simulink model "inv_im_param"  (R2026b)
settings: Solver=ode23tb  StopTime=param.sim.simlength  FixedStep=tc  MaxStep=param.glb_time.tc
values from neighbouring files (symbols this model uses):
  param = add_template_extras(param, options)    [init_model.m]
undefined symbols (not defined in the file or in its folder): magnitude
libraries: fl_lib x30, nesl_utility x13, lithium_ion_battery x1, induction_machine x1, dclink_with_center_tap x1, dead_time_generator_cmos_simulink x1, three_phase_pwm_modulator x1, three_phase_inverter_ideal_switch_based_model x1, three_phase_inverter_igbt_advanced_thermal_model x1, three_phase_inverter_mosfet_based_with_thermal_model x1, threephase_inductor_lib x1, simple_flexible_shaft x1
(part 3 of 3)

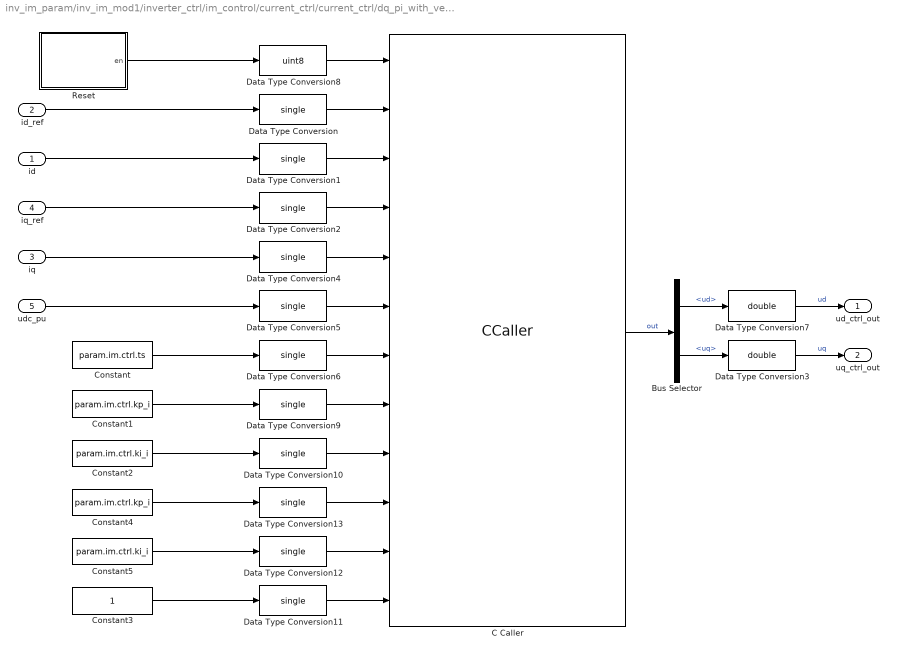
== system inv_im_param/inv_im_mod1/inverter_ctrl/im_control/current_ctrl/current_ctrl/dq_pi_with_vector_antiwindup mod1/dq_vector_pi_ccaller ==
  id : Inport
  id_ref : Inport  Port=2
  iq : Inport  Port=3
  iq_ref : Inport  Port=4
  udc_pu : Inport  Port=5
  Bus Selector : BusSelector  OutputSignals=ud,uq
  C Caller : CCaller  FunctionName=dqvector_pi_process_simulink  PortSpecificationStruct="%)30     .    ,!8   8    (     @         %    \"     T    !     0         %  0 \"0    $    _    07)G3F%M90  4&]R=$YA;64 4V-O<&4     26YD97@     5'EP90      4VEZ90      27-';&]B86P   X    P    !@    @    $          4    (     0    ,    !         !   P!O=70 #@   #     &    \"     0         !0    @    !     P    $         $  # &]U=  .    .     8    (    !          %    \"     $    &     0         0   ...(+7280 chars)"
  Constant : Constant  Value=param.im.ctrl.ts
  Constant1 : Constant  Value=param.im.ctrl.kp_i
  Constant2 : Constant  Value=param.im.ctrl.ki_i
  Constant3 : Constant
  Constant4 : Constant  Value=param.im.ctrl.kp_i
  Constant5 : Constant  Value=param.im.ctrl.ki_i
  Data Type Conversion{,1..2,4..6,9..13} (11 alike) : DataTypeConversion  OutDataTypeStr=single  SaturateOnIntegerOverflow=off  RndMeth=Floor
  Data Type Conversion3 : DataTypeConversion  OutDataTypeStr=double  SaturateOnIntegerOverflow=off  RndMeth=Floor
  Data Type Conversion7 : DataTypeConversion  OutDataTypeStr=double  SaturateOnIntegerOverflow=off  RndMeth=Floor
  Data Type Conversion8 : DataTypeConversion  OutDataTypeStr=uint8  SaturateOnIntegerOverflow=off  RndMeth=Floor
  Reset : Subsystem
  ud_ctrl_out : Outport
  uq_ctrl_out : Outport  Port=2
  wires:
  Data Type Conversion5/1 -> C Caller/6
  Data Type Conversion/1 -> C Caller/2
  C Caller/1 -> Bus Selector/1  "out"
  Data Type Conversion1/1 -> C Caller/3
  Data Type Conversion4/1 -> C Caller/5
  Data Type Conversion2/1 -> C Caller/4
  Data Type Conversion6/1 -> C Caller/7
  Bus Selector/2 -> Data Type Conversion3/1  "<uq>"
  Bus Selector/1 -> Data Type Conversion7/1  "<ud>"
  Data Type Conversion7/1 -> ud_ctrl_out/1  "ud"
  Data Type Conversion3/1 -> uq_ctrl_out/1  "uq"
  Data Type Conversion8/1 -> C Caller/1
  Data Type Conversion9/1 -> C Caller/8
  Data Type Conversion10/1 -> C Caller/9
  Data Type Conversion11/1 -> C Caller/12
  Data Type Conversion13/1 -> C Caller/10
  Data Type Conversion12/1 -> C Caller/11
  Constant3/1 -> Data Type Conversion11/1
  Constant5/1 -> Data Type Conversion12/1
  Constant4/1 -> Data Type Conversion13/1
  Constant2/1 -> Data Type Conversion10/1
  Constant1/1 -> Data Type Conversion9/1
  Constant/1 -> Data Type Conversion6/1
  udc_pu/1 -> Data Type Conversion5/1
  iq/1 -> Data Type Conversion4/1
  iq_ref/1 -> Data Type Conversion2/1
  Reset/1(en) -> Data Type Conversion8/1
  id_ref/1 -> Data Type Conversion/1
  id/1 -> Data Type Conversion1/1

== system inv_im_param/inv_im_mod1/inverter_ctrl/im_control/current_ctrl/rotor_flux_estimators/ekf/extended_kalman_observer ==
  ualphabeta : Inport
  ialphabeta : Inport  Port=2
  udc_pu : Inport  Port=3
  ekf_im : MATLAB Function  TreatAsAtomicUnit=on
  ekf_state : Scope
      settings: ActiveDisplayYMinimum=-4.1303782529271533  ActiveDisplayYMaximum=2.0916402302067323  DataLoggingVariableName=ScopeData14
  voltage_delay : Delay  DelayLength=n_delay_u
  psi_alpha_ekf_hat : Outport
  psi_beta_ekf_hat : Outport  Port=2
  phase_elec_ekf_hat : Outport  Port=3
  omega_elec_ekf_hat : Outport  Port=4
  wires:
  ualphabeta/1 -> voltage_delay/1  "u_ab_cmd"
  voltage_delay/1 -> ekf_im/1(u_ab)  "u_ab"
  ialphabeta/1 -> ekf_im/2(i_ab)  "i_ab"
  udc_pu/1 -> ekf_im/3(udc_pu)  "udc_pu"
  ekf_im/1(psi_alpha) -> psi_alpha_ekf_hat/1  "psi_alpha"
  ekf_im/2(psi_beta) -> psi_beta_ekf_hat/1  "psi_beta"
  ekf_im/3(theta) -> phase_elec_ekf_hat/1  "theta"
  ekf_im/4(omega) -> omega_elec_ekf_hat/1  "omega"
  ekf_im/5(x_hat) -> ekf_state/1  "x(k|k)"

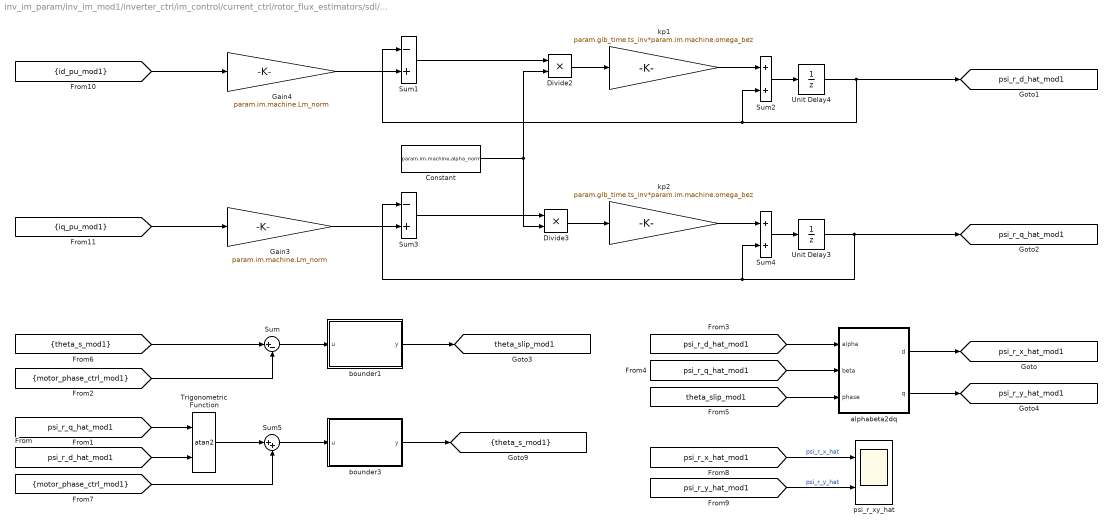
== system inv_im_param/inv_im_mod1/inverter_ctrl/im_control/current_ctrl/rotor_flux_estimators/sdl/observer_from_rotor ==
  Constant : Constant  Value=param.im.machine.alpha_norm
  Divide2 : Product
  Divide3 : Product
  Gain3 : Gain  Gain=param.im.machine.Lm_norm
  Gain4 : Gain  Gain=param.im.machine.Lm_norm
  Sum : Sum  Inputs=|+-
  Sum1 : Sum  Inputs=-+  SaturateOnIntegerOverflow=on
  Sum2 : Sum  SaturateOnIntegerOverflow=on
  Sum3 : Sum  Inputs=-+  SaturateOnIntegerOverflow=on
  Sum4 : Sum  SaturateOnIntegerOverflow=on
  Sum5 : Sum  Inputs=|++
  Trigonometric Function : Trigonometry  Operator=atan2
  Unit Delay3 : UnitDelay  SampleTime=-1
  Unit Delay4 : UnitDelay  SampleTime=-1
  alphabeta2dq : Subsystem
  bounder1 : MATLAB Function  TreatAsAtomicUnit=on
  bounder3 : MATLAB Function  TreatAsAtomicUnit=on
  kp1 : Gain  Gain=param.glb_time.ts_inv*param.im.machine.omega_bez  SaturateOnIntegerOverflow=on  OutDataTypeStr=Inherit: Same as input  ParamDataTypeStr=Inherit: Same as input
  kp2 : Gain  Gain=param.glb_time.ts_inv*param.im.machine.omega_bez  SaturateOnIntegerOverflow=on  OutDataTypeStr=Inherit: Same as input  ParamDataTypeStr=Inherit: Same as input
  psi_r_xy_hat : Scope  NumInputPorts=2
      settings: ActiveDisplayYMinimum=-0.0998429610041313  ActiveDisplayYMaximum=0.89858664903716645  DataLoggingVariableName=ScopeData10
  tag scope: psi_r_d_hat_mod1=global, psi_r_q_hat_mod1=global, psi_r_x_hat_mod1=global, psi_r_y_hat_mod1=global, theta_s_mod1=scoped, theta_slip_mod1=global
  wires:
  [psi_r_x_hat_mod1] -> psi_r_xy_hat/1  "psi_r_x_hat"
  bounder3/1(y) -> [theta_s_mod1]
  [psi_r_d_hat_mod1] -> Trigonometric Function/2
  Divide2/1 -> kp1/1
  bounder1/1(y) -> [theta_slip_mod1]
  Sum5/1 -> bounder3/1(u)
  Gain3/1 -> Sum3/2
  [psi_r_y_hat_mod1] -> psi_r_xy_hat/2  "psi_r_y_hat"
  [theta_s_mod1] -> Sum/1
  kp1/1 -> Sum2/1
  alphabeta2dq/2(q) -> [psi_r_y_hat_mod1]
  [iq_pu_mod1] -> Gain3/1
  Gain4/1 -> Sum1/2
  Unit Delay3/1 -> [psi_r_q_hat_mod1], Sum4/2, Sum3/1
  Unit Delay4/1 -> [psi_r_d_hat_mod1], Sum2/2, Sum1/1
  Divide3/1 -> kp2/1
  [theta_slip_mod1] -> alphabeta2dq/3(phase)
  Constant/1 -> Divide3/2, Divide2/2
  Sum4/1 -> Unit Delay3/1
  [motor_phase_ctrl_mod1] -> Sum/2
  Sum3/1 -> Divide3/1
  Trigonometric Function/1 -> Sum5/1
  kp2/1 -> Sum4/1
  alphabeta2dq/1(d) -> [psi_r_x_hat_mod1]
  Sum/1 -> bounder1/1(u)
  [psi_r_d_hat_mod1] -> alphabeta2dq/1(alpha)
  [id_pu_mod1] -> Gain4/1
  Sum2/1 -> Unit Delay4/1
  Sum1/1 -> Divide2/1
  [psi_r_q_hat_mod1] -> Trigonometric Function/1
  [motor_phase_ctrl_mod1] -> Sum5/2
  [psi_r_q_hat_mod1] -> alphabeta2dq/2(beta)

== system inv_im_param/inv_im_mod1/inverter_ctrl/im_control/current_ctrl/current_ctrl/dq_pi_with_vector_antiwindup mod1/dq_vector_pi/bounder1 ==
  md : Inport
  m_1 : Inport  Port=2
  m : Inport  Port=3
  Constant : Constant
  Constant1 : Constant  Value=0
  Divide : Product
  Switch : Switch  Threshold=1  SaturateOnIntegerOverflow=off  InputSameDT=off
  Switch1 : Switch  Threshold=1  SaturateOnIntegerOverflow=off  InputSameDT=off
  md_sat : Outport  VectorParamsAs1DForOutWhenUnconnected=off
  clip : Outport  Port=2  VectorParamsAs1DForOutWhenUnconnected=off
  wires:
  md/1 -> Switch1/3, Divide/2
  m_1/1 -> Divide/1
  Divide/1 -> Switch1/1
  Switch1/1 -> md_sat/1
  Switch/1 -> clip/1
  m/1 -> Switch/2, Switch1/2
  Constant/1 -> Switch/1
  Constant1/1 -> Switch/3

== system inv_im_param/inv_im_mod1/inverter_ctrl/im_control/current_ctrl/current_ctrl/dq_pi_with_vector_antiwindup mod1/dq_vector_pi/bounder2 ==
  m : Inport
  m_1 : Inport  Port=2
  mq : Inport  Port=3
  Constant : Constant
  Constant1 : Constant  Value=0
  Divide : Product
  Switch : Switch  Threshold=1  SaturateOnIntegerOverflow=off  InputSameDT=off
  Switch1 : Switch  Threshold=1  SaturateOnIntegerOverflow=off  InputSameDT=off
  mq_sat : Outport  VectorParamsAs1DForOutWhenUnconnected=off
  clip : Outport  Port=2  VectorParamsAs1DForOutWhenUnconnected=off
  wires:
  Constant1/1 -> Switch/3
  Constant/1 -> Switch/1
  m/1 -> Switch1/2, Switch/2
  Switch/1 -> clip/1
  Switch1/1 -> mq_sat/1
  Divide/1 -> Switch1/1
  m_1/1 -> Divide/1
  mq/1 -> Divide/2, Switch1/3

== system inv_im_param/inv_im_mod1/inverter_ctrl/im_control/current_ctrl/current_ctrl/dq_pi_with_vector_antiwindup mod1/dq_vector_pi/pi_d ==
  id_tilde : Inport
  clip : Inport  Port=2
  1/Ti : Gain  Gain=param.im.ctrl.kp_i  SaturateOnIntegerOverflow=on  OutDataTypeStr=Inherit: Same as input  ParamDataTypeStr=Inherit: Same as input
  Constant : Constant  Value=0
  Sum2 : Sum  Inputs=+-  SaturateOnIntegerOverflow=on
  Sum4 : Sum  SaturateOnIntegerOverflow=on
  Sum5 : Sum  SaturateOnIntegerOverflow=on
  Switch1 : Switch  Threshold=0.5  SaturateOnIntegerOverflow=off  InputSameDT=off
  Switch2 : Switch  Threshold=0.5  SaturateOnIntegerOverflow=off  InputSameDT=off
  Unit Delay1 : UnitDelay  SampleTime=-1
  Unit Delay2 : UnitDelay  SampleTime=-1
  kp1 : Gain  Gain=param.ctrl.CTRPIFF_CLIP_RELEASE*param.glb_time.ts_inv  SaturateOnIntegerOverflow=on  OutDataTypeStr=Inherit: Same as input  ParamDataTypeStr=Inherit: Same as input
  kp2 : Gain  Gain=param.im.ctrl.ki_i*param.glb_time.ts_inv  SaturateOnIntegerOverflow=on  OutDataTypeStr=Inherit: Same as input  ParamDataTypeStr=Inherit: Same as input
  ud_out : Outport  VectorParamsAs1DForOutWhenUnconnected=off
  wires:
  id_tilde/1 -> kp2/1, 1/Ti/1
  Sum5/1 -> ud_out/1
  Switch1/1 -> Unit Delay2/1
  Sum4/1 -> Sum5/2, Switch1/3
  kp1/1 -> Sum2/2
  Sum2/1 -> Switch1/1
  Unit Delay2/1 -> Sum4/2, kp1/1, Sum2/1
  1/Ti/1 -> Sum5/1
  Switch2/1 -> Sum4/1
  kp2/1 -> Switch2/3
  clip/1 -> Unit Delay1/1
  [clip] -> Switch2/2
  [clip] -> Switch1/2
  Constant/1 -> Switch2/1
  Unit Delay1/1 -> [clip]

== system inv_im_param/inv_im_mod1/inverter_ctrl/im_control/current_ctrl/current_ctrl/dq_pi_with_vector_antiwindup mod1/dq_vector_pi/pi_q ==
  iq_tilde : Inport
  clip : Inport  Port=2
  1/Ti : Gain  Gain=param.im.ctrl.kp_i  SaturateOnIntegerOverflow=on  OutDataTypeStr=Inherit: Same as input  ParamDataTypeStr=Inherit: Same as input
  Constant : Constant  Value=0
  Sum2 : Sum  Inputs=+-  SaturateOnIntegerOverflow=on
  Sum4 : Sum  SaturateOnIntegerOverflow=on
  Sum5 : Sum  SaturateOnIntegerOverflow=on
  Switch1 : Switch  Threshold=0.5  SaturateOnIntegerOverflow=off  InputSameDT=off
  Switch2 : Switch  Threshold=0.5  SaturateOnIntegerOverflow=off  InputSameDT=off
  Unit Delay1 : UnitDelay  SampleTime=-1
  Unit Delay2 : UnitDelay  SampleTime=-1
  kp1 : Gain  Gain=param.ctrl.CTRPIFF_CLIP_RELEASE*param.glb_time.ts_inv  SaturateOnIntegerOverflow=on  OutDataTypeStr=Inherit: Same as input  ParamDataTypeStr=Inherit: Same as input
  kp2 : Gain  Gain=param.im.ctrl.ki_i*param.glb_time.ts_inv  SaturateOnIntegerOverflow=on  OutDataTypeStr=Inherit: Same as input  ParamDataTypeStr=Inherit: Same as input
  Vqs_out : Outport  VectorParamsAs1DForOutWhenUnconnected=off
  wires:
  Constant/1 -> Switch2/1
  [clip] -> Switch1/2
  [clip] -> Switch2/2
  clip/1 -> Unit Delay1/1
  kp2/1 -> Switch2/3
  Switch2/1 -> Sum4/1
  1/Ti/1 -> Sum5/1
  Unit Delay2/1 -> Sum2/1, kp1/1, Sum4/2
  Sum2/1 -> Switch1/1
  kp1/1 -> Sum2/2
  Sum4/1 -> Sum5/2, Switch1/3
  Switch1/1 -> Unit Delay2/1
  iq_tilde/1 -> 1/Ti/1, kp2/1
  Unit Delay1/1 -> [clip]
  Sum5/1 -> Vqs_out/1

== system inv_im_param/inv_im_mod1/inverter_ctrl/im_control/current_ctrl/current_ctrl/dq_pi_with_vector_antiwindup mod1/dq_vector_pi/switch ==
  clip 1 : Inport
  clip 2 : Inport  Port=2
  Constant4 : Constant
  Constant5 : Constant  Value=0
  Sum1 : Sum  SaturateOnIntegerOverflow=on
  Switch : Switch  Threshold=0.5  SaturateOnIntegerOverflow=off  InputSameDT=off
  clip : Outport  VectorParamsAs1DForOutWhenUnconnected=off
  wires:
  Constant5/1 -> Switch/3
  Switch/1 -> clip/1
  Constant4/1 -> Switch/1
  Sum1/1 -> Switch/2
  clip 1/1 -> Sum1/1
  clip 2/1 -> Sum1/2

== system inv_im_param/inv_im_mod1/inverter_ctrl/im_control/current_ctrl/current_ctrl/dq_pi_with_vector_antiwindup mod1/dq_vector_pi/vector lenght ==
  md : Inport
  mq : Inport  Port=2
  Math Function : Math  Operator=magnitude^2  SignedPower=on
  Math Function1 : Math  Operator=magnitude^2  SignedPower=on
  Math Function2 : Math  Operator=reciprocal  SignedPower=on
  Sqrt : Sqrt
  Sum5 : Sum  SaturateOnIntegerOverflow=on
  m_1 : Outport  VectorParamsAs1DForOutWhenUnconnected=off
  m : Outport  Port=2  VectorParamsAs1DForOutWhenUnconnected=off
  wires:
  Sqrt/1 -> m/1, Math Function2/1
  mq/1 -> Math Function1/1
  Math Function1/1 -> Sum5/2
  Math Function/1 -> Sum5/1
  Sum5/1 -> Sqrt/1
  Math Function2/1 -> m_1/1
  md/1 -> Math Function/1

== system inv_im_param/inv_im_mod1/inverter_ctrl/im_control/current_ctrl/current_ctrl/dq_pi_with_vector_antiwindup mod1/dq_vector_pi_ccaller/Reset ==
  Step : Step  Time=0.05  InitialValue=1  FinalValue=0
  en : Outport
  wires:
  Step/1 -> en/1

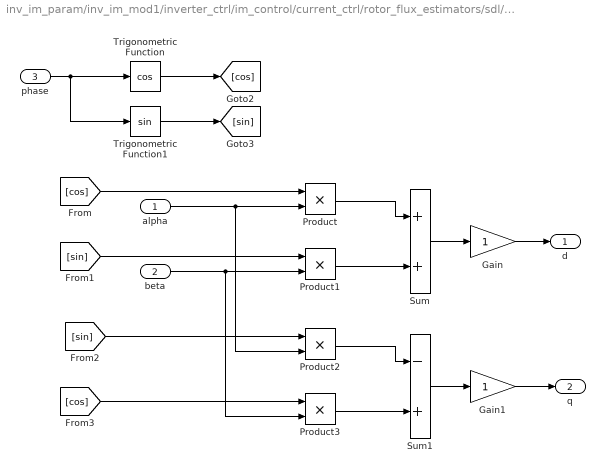
== system inv_im_param/inv_im_mod1/inverter_ctrl/im_control/current_ctrl/rotor_flux_estimators/sdl/observer_from_rotor/alphabeta2dq ==
  alpha : Inport
  beta : Inport  Port=2
  phase : Inport  Port=3
  Gain : Gain
  Gain1 : Gain
  Product{,1..3} (4 alike) : Product  RndMeth=Zero
  Sum : Sum
  Sum1 : Sum  Inputs=-+
  Trigonometric Function : Trigonometry  Operator=cos
  Trigonometric Function1 : Trigonometry
  d : Outport  VectorParamsAs1DForOutWhenUnconnected=off
  q : Outport  Port=2  VectorParamsAs1DForOutWhenUnconnected=off
  wires:
  [cos] -> Product/1
  alpha/1 -> Product/2, Product2/2
  Product/1 -> Sum/1
  Product1/1 -> Sum/2
  [sin] -> Product1/1
  beta/1 -> Product1/2, Product3/2
  Sum/1 -> Gain/1
  [sin] -> Product2/1
  Product2/1 -> Sum1/1
  Product3/1 -> Sum1/2
  [cos] -> Product3/1
  Sum1/1 -> Gain1/1
  Gain/1 -> d/1
  Gain1/1 -> q/1
  Trigonometric Function1/1 -> [sin]
  Trigonometric Function/1 -> [cos]
  phase/1 -> Trigonometric Function/1, Trigonometric Function1/1

== matlab function inv_im_param/inv_im_mod1/inverter_ctrl/im_control/current_ctrl/uvw2dq/uvw2alphabeta ==
  data: u input; alpha output; v input; w input; beta output
function [alpha,beta] = uvw2alphabeta(u,v,w)

alpha = 2/3*(u - 1/2*v - 1/2*w);
beta  = 2/3*(sqrt(3)/2*(v - w));

end

== matlab function inv_im_param/inv_im_mod1/inverter_ctrl/im_control/current_ctrl/us xy2dq/xy2dq ==
  data: d input; alpha output; q input; gamma input; beta output
function [alpha,beta] = dq2alphabeta(d,q,gamma)

    alpha  =  d*cos(gamma) - q*sin(gamma);
    beta = d*sin(gamma) + q*cos(gamma);

end

== matlab function inv_im_param/inv_im_mod1/inverter_ctrl/im_control/current_ctrl/rotor_flux_estimators/sdl/xy2dq1 ==
  data: d input; alpha output; q input; gamma input; beta output
function [alpha,beta] = dq2alphabeta(d,q,gamma)

    alpha  =  d*cos(gamma) - q*sin(gamma);
    beta = d*sin(gamma) + q*cos(gamma);

end

== matlab function inv_im_param/inv_im_mod1/inverter_ctrl/im_control/current_ctrl/rotor_flux_estimators/sdl/observer_from_rotor/bounder3 ==
  data: u input; y output
function y = bounder(u)
    
    y = -pi + mod(u+3*pi,2*pi);
    
end

== matlab function inv_im_param/inv_im_mod1/inverter_ctrl/im_control/current_ctrl/rotor_flux_estimators/sdl/observer_from_rotor/bounder1 ==
  data: u input; y output
function y = bounder(u)
    
    y = -pi + mod(u+3*pi,2*pi);
    
end

== matlab function inv_im_param/inv_im_mod1/inverter_ctrl/im_control/encoder-sensorless-switch/double_integrator_observer/bounder1 ==
  data: u input; y output
function y = bounder(u)
    y = -pi + mod(u+3*pi,2*pi);
end

== matlab function inv_im_param/inv_im_mod1/inverter_ctrl/im_control/encoder-sensorless-switch/double_integrator_observer/bounder2 ==
  data: u input; y output
function y = bounder(u)
    y = -pi + mod(u+3*pi,2*pi);
end

== matlab function inv_im_param/inv_im_mod1/inverter_ctrl/im_control/current_ctrl/rotor_flux_estimators/ekf/extended_kalman_observer/ekf_im ==
  data: u_ab input; i_ab input; udc_pu input; psi_alpha output; psi_beta output; theta output; omega output; x_hat output; ts parameter; omega_b parameter; sigma_n parameter; rs_n parameter; lm_n parameter; lr_n parameter; alpha_n parameter; kr parameter; tau_m parameter; q_diag parameter; r_diag parameter; p0_diag parameter; x0 parameter; n_hold parameter; cov_order parameter
function [psi_alpha, psi_beta, theta, omega, x_hat] = ekf_im(u_ab, i_ab, udc_pu, ts, omega_b, sigma_n, rs_n, lm_n, lr_n, alpha_n, kr, tau_m, q_diag, r_diag, p0_diag, x0, n_hold, cov_order)
% Extended Kalman filter of the induction machine: rotor flux, speed and load torque from the
% voltage command and the measured current. One call per control period; the algorithm is
% ekf_im_step of the library (user_defined_functions/ekf_im), the parameters come from
% ekf_im_setup (param.im.ctrl.ekf) through the mask of extended_kalman_observer.
% States x = [i_alpha; i_beta; psi_alpha; psi_beta; omega; T_load], pu of the machine bases.
%
%   u_ab    voltage command [u_alpha; u_beta] times u_im_scale_ekf, delayed by n_delay_u steps
%           (Delay block in front): the voltage applied between the sampling instants of the
%           previous and of the present current measurement, per pu of DC-link voltage
%   i_ab    measured stator current [i_alpha; i_beta] in pu of ibez
%   udc_pu  measured DC-link voltage in pu of param.afe.hw.udc_nom: the inverter applies the
%           command as a fraction of the DC-link voltage
%
%   psi_alpha, psi_beta  estimated rotor flux [pu]
%   theta                rotor flux angle [rad]
%   omega                estimated electrical rotor speed [pu]
%   x_hat                whole estimate (scope ekf_state)

persistent x P k
if isempty(x)
    x = x0(:);
    P = diag(p0_diag(:));
    k = 0;
end

e = struct('ts', ts, 'omega_b', omega_b, 'sigma_n', sigma_n, 'rs_n', rs_n, 'lm_n', lm_n, ...
           'lr_n', lr_n, 'alpha_n', alpha_n, 'kr', kr, 'tau_m', tau_m, 'q_diag', q_diag(:), ...
           'r_diag', r_diag(:), 'p0_diag', p0_diag(:), 'cov_order', cov_order);

% the first n_hold samples are the magnetization at standstill: speed and load torque held at zero
standstill = k < n_hold;
if standstill
    k = k + 1;
end

[x, P] = ekf_im_step(x, P, u_ab(:)*udc_pu, i_ab(:), standstill, e);

psi_alpha = x(3);
psi_beta = x(4);
theta = atan2(x(4), x(3));
omega = x(5);
x_hat = x;
end

== matlab function inv_im_param/inv_im_mod1/inverter_ctrl/im_control/current_ctrl/is uvw2xy/alphabeta2dq ==
  data: alpha input; d output; beta input; gamma input; q output
function [d,q] = alphabeta2dq(alpha,beta,gamma)

    d  =  alpha*cos(gamma) + beta*sin(gamma);
    q = -alpha*sin(gamma) + beta*cos(gamma);

end

== matlab function inv_im_param/inv_im_mod1/inverter_ctrl/im_control/current_ctrl/is uvw2xy/uvw2alphabeta ==
  data: u input; alpha output; v input; w input; beta output
function [alpha,beta] = uvw2alphabeta(u,v,w)

alpha = 2/3*(u - 1/2*v - 1/2*w);
beta  = 2/3*(sqrt(3)/2*(v - w));

end

== matlab function inv_im_param/inv_im_mod1/inverter_ctrl/im_control/current_ctrl/us xy2alphabeta/xy2dq ==
  data: d input; alpha output; q input; gamma input; beta output
function [alpha,beta] = dq2alphabeta(d,q,gamma)

    alpha  =  d*cos(gamma) - q*sin(gamma);
    beta = d*sin(gamma) + q*cos(gamma);

end

== matlab function inv_im_param/motor_load_setting/bounder1 ==
  data: u input; y output
function y = bounder(u)
    y = -pi + mod(u+3*pi,2*pi);
end

== matlab function inv_im_param/inv_im_mod1/inverter_ctrl/im_control/current_ctrl/uvw2dq/alphabeta2dq ==
  data: alpha input; d output; beta input; gamma input; q output
function [d,q] = alphabeta2dq(alpha,beta,gamma)

    d  =  alpha*cos(gamma) + beta*sin(gamma);
    q = -alpha*sin(gamma) + beta*cos(gamma);

end

== matlab function inv_im_param/inv_im_mod1/inverter_ctrl/im_control/current_ctrl/rotor_flux_estimators/sdl/xy2dq ==
  data: d input; alpha output; q input; gamma input; beta output
function [alpha,beta] = dq2alphabeta(d,q,gamma)

    alpha  =  d*cos(gamma) - q*sin(gamma);
    beta = d*sin(gamma) + q*cos(gamma);

end
